simulink model "multifoc"  (R2025b)
settings: Solver=FixedStepAuto  StartTime=0.0  StopTime=inf  RelTol=1e-3
model workspace (MAT data in the model file):
  idx = Simulink.Parameter
  idx.Value = 15
  idx.Complexity = 'real'
  idx.Dimensions = [1 1]
  idx.DataType = 'auto'
undefined symbols (not defined in the file): AmcfocInitConf, ControlModes, EventTypes, externals, motor_id
libraries: simulink x4, dspsigops x2
settings Model: DataDictionary=amcfoc.sldd  SimulationMode=accelerator  Creator=mfussi  LastModifiedBy=rpumpo
settings SolverCC: ConcurrentTasks=on  AutoInsertRateTranBlk=on
settings DataIOCC: SaveOutput=off  DSMLogging=off  SaveTime=off
settings OptimizationCC: SimCompilerOptimization=on
settings RTWCC: GPUComputeCapability=3.5

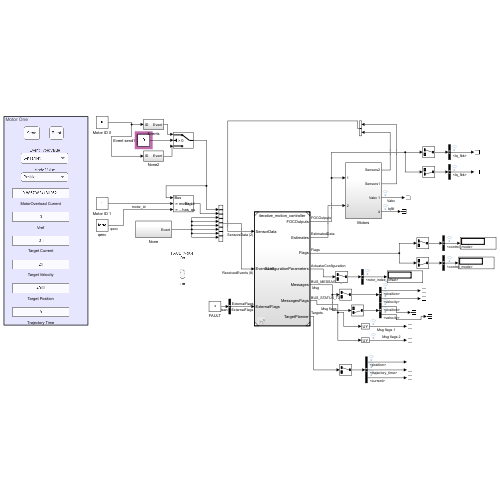
[thumbnail: Simulink's stored preview of the top-level diagram]
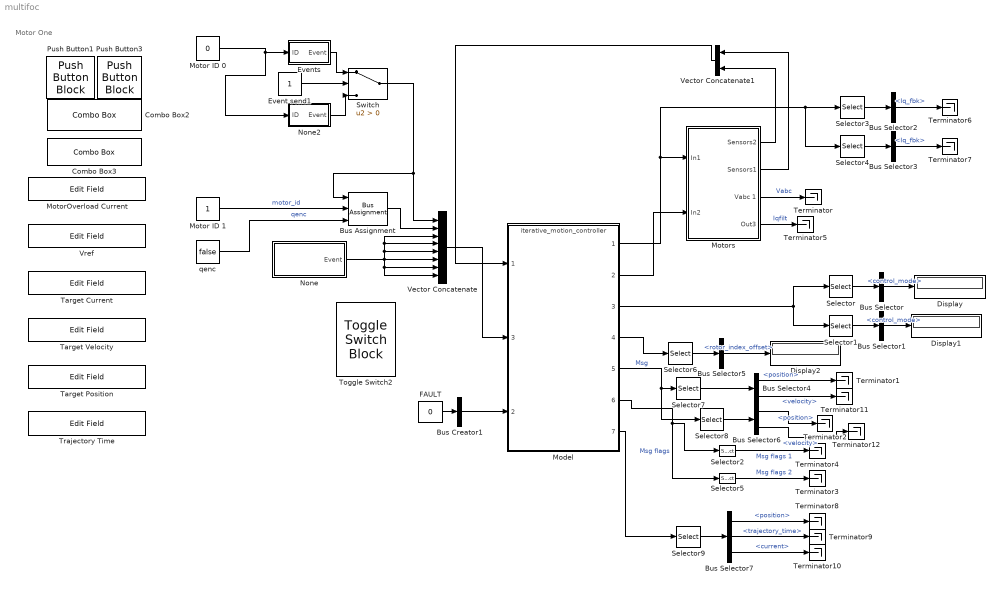
== system multifoc ==
  note: Motor One
  Bus Assignment : BusAssignment  AssignedSignals=motor_id,externals.has_quadrature_encoder
  Bus Creator1 : BusCreator  Inputs=1  OutDataTypeStr=Bus: ExternalFlags  NonVirtualBus=on
      settings: InheritFromInputs=off
  Bus Selector : BusSelector  OutputSignals=control_mode
  Bus Selector1 : BusSelector  OutputSignals=control_mode
  Bus Selector2 : BusSelector  OutputSignals=Iq_fbk
  Bus Selector3 : BusSelector  OutputSignals=Iq_fbk
  Bus Selector4 : BusSelector  OutputSignals=foc.position,foc.velocity
  Bus Selector5 : BusSelector  OutputSignals=motor.externals.rotor_index_offset
  Bus Selector6 : BusSelector  OutputSignals=foc.position,foc.velocity
  Bus Selector7 : BusSelector  OutputSignals=position,trajectory_time,current
  Combo Box2 : ComboBox  SelectedLabel=SetTarget  UseEnumeratedDataType=on  EnumeratedDataType=EventTypes
  Combo Box3 : ComboBox  SelectedLabel=Position  UseEnumeratedDataType=on  EnumeratedDataType=ControlModes
  Display : Display
  Display1 : Display
  Display2 : Display
  Event send1 : Constant
  Events : Subsystem
  FAULT : Constant  Value=0  OutDataTypeStr=Inherit: Inherit via back propagation
  Model : ModelReference  ModelNameDialog=iterative_motion_controller.slx  SimulationMode=Normal  ModelReferenceVersion=5.18
      settings: PortSchema="{\"entries\":[{\"content\":{\"sides\":[{\"content\":{\"connectorIds\":[\"In1\",\"In3\",\"In2\"]},\"type\":\"ConnectorPlacement.EquallySpacedRectSide\",\"uuid\":\"934c1d33-4450-4a0d-b709-1a42a1f76a8a\"},{\"content\":{\"connectorIds\":[\"Out1\",\"Out2\",\"Out3\",\"Out4\",\"Out5\",\"Out6\",\"Out7\"],\"side\":\"RIGHT\"},\"type\":\"ConnectorPlacement.EquallySpacedRectSide\",\"uuid\":\"07cc3f64-4a6c-4a49-ab3b-6bdd8946d703\"},{\"content\":{\"side\":\"TOP\"},\"type\":\"ConnectorPlacement.EquallySpacedRectSide\",\"uuid\":\"bdfb7dfb-875f-4552-909e-d1a15bca8e36\"}]},\"type\":\"ConnectorPlacement.EquallySpacedConnector\",\"uuid\":\"d809c882-6d9c-4cbc-bba4-fc08c365081a\"}],\"packageUris\":[\"http://schema.mathworks.com/mf0/Connector/R2020b\"],\"version\":\"1.0\"}"
  Motor ID 0 : Constant  Value=0  OutDataTypeStr=Inherit: Inherit via back propagation
  Motor ID 1 : Constant  OutDataTypeStr=Inherit: Inherit via back propagation
  MotorOverload Current : EditField  LabelPosition=Hide  ShowInitialText=on  Alignment=Center
  Motors : Subsystem
  None : Subsystem
  None2 : Subsystem
  Push Button1 : PushButtonBlock  ButtonText=Send  IconOnColor=[0.0, 0.39215686274509803, 0.0]  IconOffColor=[0.0, 1.0, 0.0]  OffValue=0.000000
  Push Button3 : PushButtonBlock  ButtonText=Burst  ButtonType=Latch  IconOnColor=[0.0, 0.39215686274509803, 0.0]  IconOffColor=[0.0, 1.0, 0.0]  OffValue=0.000000
  Selector{,2..3,6..7,9} (6 alike) : Selector  InputPortWidth=2  IndexOptions=Index vector (dialog)  Indices=1  OutputSizes=1
  Selector{1,4..5,8} (4 alike) : Selector  InputPortWidth=2  IndexOptions=Index vector (dialog)  Indices=2  OutputSizes=1
  Switch : Switch  Criteria=u2 > Threshold  SaturateOnIntegerOverflow=off  InputSameDT=off
  Target Current : EditField  LabelPosition=Hide  ShowInitialText=on  Alignment=Center
  Target Position : EditField  LabelPosition=Hide  ShowInitialText=on  Alignment=Center
  Target Velocity : EditField  LabelPosition=Hide  ShowInitialText=on  Alignment=Center
  Terminator{,1..12} (13 alike) : Terminator
  Toggle Switch2 : ToggleSwitchBlock
  Trajectory Time : EditField  LabelPosition=Hide  ShowInitialText=on  Alignment=Center
  Vector Concatenate : Concatenate  NumInputs=8
  Vector Concatenate1 : Concatenate
  Vref : EditField  LabelPosition=Hide  ShowInitialText=on  Alignment=Center
  qenc : Constant  Value=false  OutDataTypeStr=boolean
  wires:
  Event send1/1 -> Switch/2
  None/1(Event) -> Vector Concatenate/3, Vector Concatenate/4, Vector Concatenate/5, Vector Concatenate/8, Vector Concatenate/7, Vector Concatenate/6
  FAULT/1 -> Bus Creator1/1
  Bus Creator1/1 -> Model/2
  Vector Concatenate1/1 -> Model/1
  Motors/2(Sensors1) -> Vector Concatenate1/1
  Motors/3(Vabc 1) -> Terminator/1  "Vabc"
  Motors/4(Out3) -> Terminator5/1  "Iqfilt"
  Selector/1 -> Bus Selector/1
  Selector1/1 -> Bus Selector1/1
  Bus Selector/1 -> Display/1  "<control_mode>"
  Bus Selector1/1 -> Display1/1  "<control_mode>"
  Motors/1(Sensors2) -> Vector Concatenate1/2
  Model/1 -> Selector4/1, Selector3/1, Motors/1(In1)
  Bus Selector2/1 -> Terminator6/1  "<Iq_fbk>"
  Bus Selector3/1 -> Terminator7/1  "<Iq_fbk>"
  Selector4/1 -> Bus Selector3/1
  Selector3/1 -> Bus Selector2/1
  Model/2 -> Motors/2(In2)
  Model/6 -> Selector2/1, Selector5/1  "Msg flags"
  Model/5 -> Selector8/1, Selector7/1  "Msg"
  Selector5/1 -> Terminator3/1  "Msg flags 2"
  Selector2/1 -> Terminator4/1  "Msg flags 1"
  Motor ID 1/1 -> Bus Assignment/2  "motor_id"
  Motor ID 0/1 -> Events/1(ID), None2/1(ID)
  qenc/1 -> Bus Assignment/3  "qenc"
  Model/3 -> Selector/1, Selector1/1
  Model/4 -> Selector6/1
  Selector6/1 -> Bus Selector5/1
  Bus Selector5/1 -> Display2/1  "<rotor_index_offset>"
  Selector7/1 -> Bus Selector4/1
  Selector8/1 -> Bus Selector6/1
  Bus Selector4/1 -> Terminator1/1  "<position>"
  Bus Selector6/1 -> Terminator2/1  "<position>"
  Model/7 -> Selector9/1
  Selector9/1 -> Bus Selector7/1
  Bus Selector7/1 -> Terminator8/1  "<position>"
  Bus Selector7/2 -> Terminator9/1  "<trajectory_time>"
  Vector Concatenate/1 -> Model/3
  Events/1(Event) -> Switch/1
  Bus Selector7/3 -> Terminator10/1  "<current>"
  None2/1(Event) -> Switch/3
  Switch/1 -> Vector Concatenate/1, Bus Assignment/1
  Bus Assignment/1 -> Vector Concatenate/2
  Bus Selector4/2 -> Terminator11/1  "<velocity>"
  Bus Selector6/2 -> Terminator12/1  "<velocity>"

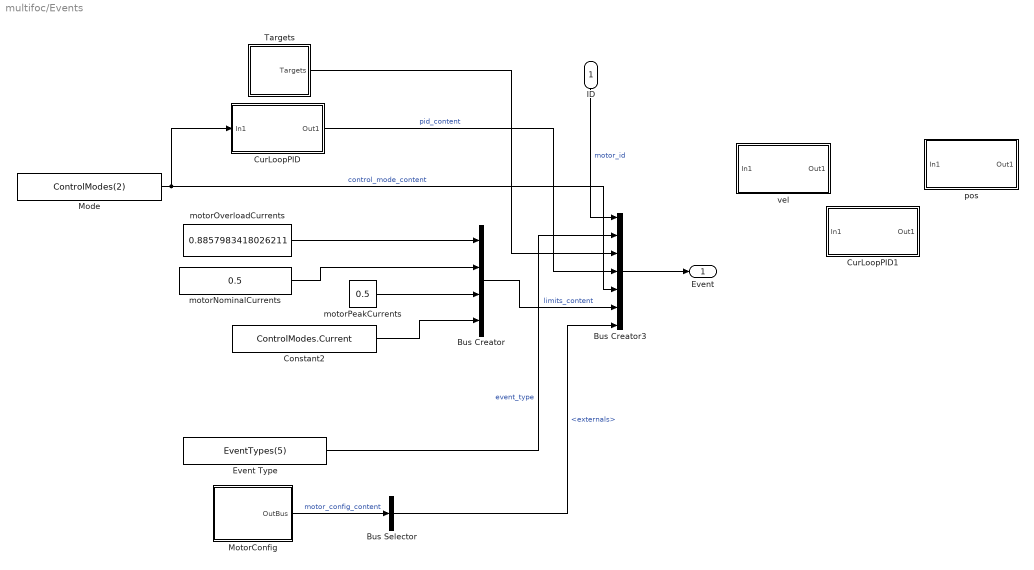
== system multifoc/Events ==
  ID : Inport
  Bus Creator : BusCreator  Inputs=4  OutDataTypeStr=Bus: SupervisorInputLimits
  Bus Creator3 : BusCreator  Inputs=7  OutDataTypeStr=Bus: ReceivedEvents  NonVirtualBus=on
  Bus Selector : BusSelector  OutputSignals=externals
  Constant2 : Constant  Value=ControlModes.Current  OutDataTypeStr=Enum: ControlModes
  CurLoopPID : Subsystem  mask{OutMax=3, OutMin=-3, P=10, I=10, D=0, N=0, I0=0, D0=0, shift_factor=0}
      mask prompts: shift_factor "Shift Factor"
  CurLoopPID1 : Subsystem  mask{OutMax=0, OutMin=0, P=2, I=500, D=0, N=10, I0=0, D0=0, shift_factor=0}
      mask prompts: shift_factor "Shift Factor"
  Event Type : Constant  Value=EventTypes(5)  OutDataTypeStr=Enum: EventTypes
  Mode : Constant  Value=ControlModes(2)  OutDataTypeStr=Enum: ControlModes
  MotorConfig : Subsystem  mask{has_hall_sens=AmcfocInitConf(1).motor.externals.has_hall_sens, has_quadrature_encoder=false, has_speed_quadrature_encoder=AmcfocInitConf(1).motor.externals.has_speed_quadrature_encoder, has_torque_sens=AmcfocInitConf(1).motor.externals.has_temperature_sens, use_index=false, enable_verbosity=AmcfocInitConf(1).motor.externals.enable_verbosity, hall_sensors_offset=0, rotor_encoder_resolution=1, rotor_index_offset=AmcfocInitConf(1).motor.externals.rotor_index_offset, encoder_tolerance=AmcfocInitConf(1).motor.externals.encoder_tolerance, pole_pairs=AmcfocInitConf(1).motor.externals.pole_pairs, reduction=100, Kbemf=AmcfocInitConf(1).motor.Kbemf, Rphase=AmcfocInitConf(1).motor.Rphase, Imin=AmcfocInitConf(1).motor.Imin, Imax=AmcfocInitConf(1).motor.Imax, Vmax=AmcfocInitConf(1).motor.Vmax, R=AmcfocInitConf(1).motor.resistance, L=AmcfocInitConf(1).motor.inductance, Rt=AmcfocInitConf(1).motor.thermal_resistance, tau=AmcfocInitConf(1).motor.thermal_time_constant}
      mask prompts: R "Motor Resistance"; L "Motor Inductance"; Rt "Thermal Resistance"; tau "Thermal Time Constant"
  Targets : Subsystem
  motorNominalCurrents : Constant  Value=0.5  OutDataTypeStr=single
  motorOverloadCurrents : Constant  Value=0.8857983418026211  OutDataTypeStr=single
  motorPeakCurrents : Constant  Value=0.5  OutDataTypeStr=single
  pos : Subsystem  mask{OutMax=0, OutMin=0, P=2, I=500, D=0, N=10, I0=0, D0=0, shift_factor=0}
      mask prompts: shift_factor "Shift Factor"
  vel : Subsystem  mask{OutMax=0, OutMin=0, P=2, I=500, D=0, N=10, I0=0, D0=0, shift_factor=0}
      mask prompts: shift_factor "Shift Factor"
  Event : Outport  OutDataTypeStr=Bus: ReceivedEvents
  wires:
  Bus Creator/1 -> Bus Creator3/6  "limits_content"
  Bus Selector/1 -> Bus Creator3/7  "<externals>"
  Mode/1 -> Bus Creator3/5, CurLoopPID/1(In1)  "control_mode_content"
  Event Type/1 -> Bus Creator3/2  "event_type"
  CurLoopPID/1(Out1) -> Bus Creator3/4  "pid_content"
  motorPeakCurrents/1 -> Bus Creator/3
  Constant2/1 -> Bus Creator/4
  motorOverloadCurrents/1 -> Bus Creator/1
  motorNominalCurrents/1 -> Bus Creator/2
  Bus Creator3/1 -> Event/1
  ID/1 -> Bus Creator3/1  "motor_id"
  MotorConfig/1(OutBus) -> Bus Selector/1  "motor_config_content"
  Targets/1(Targets) -> Bus Creator3/3

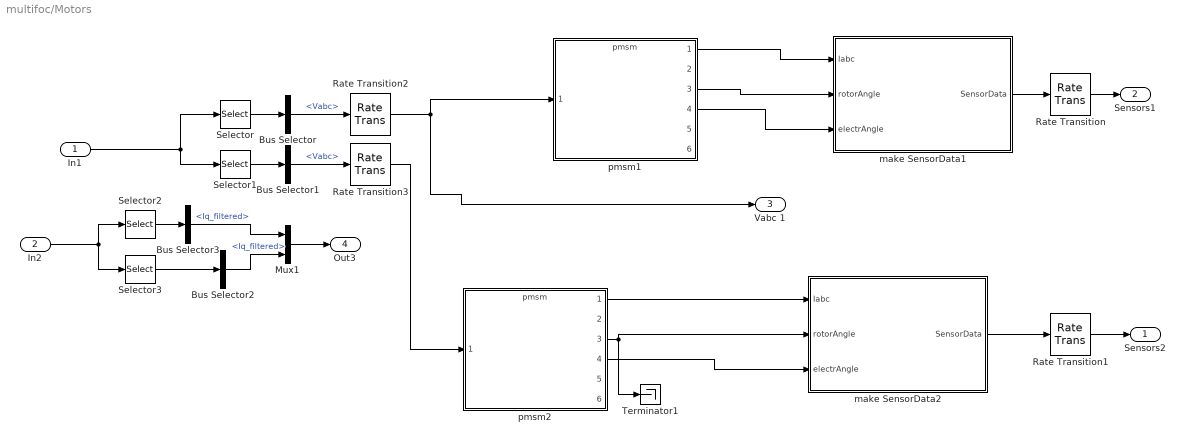
== system multifoc/Motors ==
  In1 : Inport
  In2 : Inport  Port=2
  Bus Selector : BusSelector  OutputSignals=Vabc
  Bus Selector1 : BusSelector  OutputSignals=Vabc
  Bus Selector2 : BusSelector  OutputSignals=Iq_filtered
  Bus Selector3 : BusSelector  OutputSignals=Iq_filtered
  Mux1 : Mux  Inputs=2
  Rate Transition : RateTransition  Integrity=off  OutPortSampleTime=Ts_ControlFOC
  Rate Transition1 : RateTransition  Integrity=off  OutPortSampleTime=Ts_ControlFOC
  Rate Transition2 : RateTransition  Integrity=off
  Rate Transition3 : RateTransition  Integrity=off
  Selector : Selector  InputPortWidth=2  IndexOptions=Index vector (dialog)  Indices=1  OutputSizes=1
  Selector1 : Selector  InputPortWidth=2  IndexOptions=Index vector (dialog)  Indices=2  OutputSizes=1
  Selector2 : Selector  InputPortWidth=2  IndexOptions=Index vector (dialog)  Indices=1  OutputSizes=1
  Selector3 : Selector  InputPortWidth=2  IndexOptions=Index vector (dialog)  Indices=2  OutputSizes=1
  Terminator1 : Terminator
  make SensorData1 : Subsystem
  make SensorData2 : Subsystem
  pmsm1 : ModelReference  ModelNameDialog=pmsm.slx  SimulationMode=Normal  ModelReferenceVersion=10.6  OutputSignalHandling=Zero-order hold
  pmsm2 : ModelReference  ModelNameDialog=pmsm.slx  SimulationMode=Normal  ModelReferenceVersion=10.6
  Sensors2 : Outport
  Sensors1 : Outport  Port=2
  Vabc 1 : Outport  Port=3
  Out3 : Outport  Port=4
  wires:
  pmsm2/1 -> make SensorData2/1(Iabc)
  Bus Selector1/1 -> Rate Transition3/1  "<Vabc>"
  make SensorData1/1(SensorData) -> Rate Transition/1
  Selector3/1 -> Bus Selector2/1
  pmsm2/3 -> make SensorData2/2(rotorAngle), Terminator1/1
  pmsm1/1 -> make SensorData1/1(Iabc)
  In2/1 -> Selector2/1, Selector3/1
  Bus Selector/1 -> Rate Transition2/1  "<Vabc>"
  Selector/1 -> Bus Selector/1
  Selector1/1 -> Bus Selector1/1
  Selector2/1 -> Bus Selector3/1
  Rate Transition2/1 -> pmsm1/1, Vabc 1/1
  Mux1/1 -> Out3/1
  make SensorData2/1(SensorData) -> Rate Transition1/1
  In1/1 -> Selector1/1, Selector/1
  Bus Selector3/1 -> Mux1/1  "<Iq_filtered>"
  Bus Selector2/1 -> Mux1/2  "<Iq_filtered>"
  Rate Transition/1 -> Sensors1/1
  Rate Transition1/1 -> Sensors2/1
  Rate Transition3/1 -> pmsm2/1
  pmsm1/3 -> make SensorData1/2(rotorAngle)
  pmsm1/4 -> make SensorData1/3(electrAngle)
  pmsm2/4 -> make SensorData2/3(electrAngle)

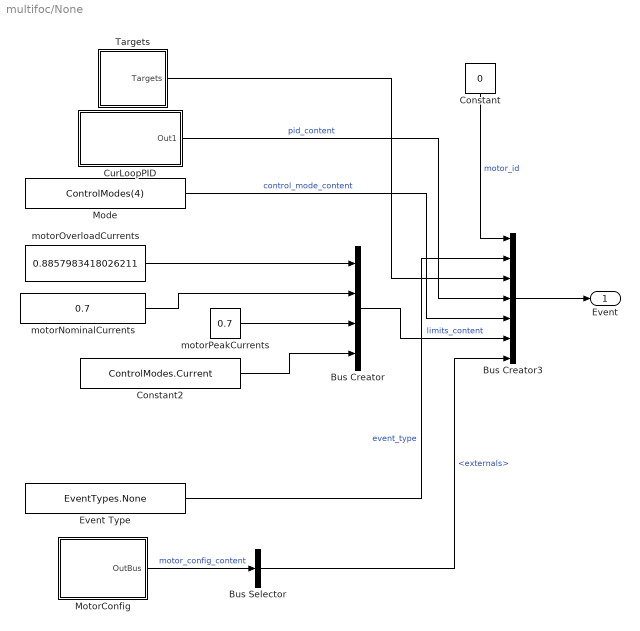
== system multifoc/None ==
  Bus Creator : BusCreator  Inputs=4  OutDataTypeStr=Bus: SupervisorInputLimits
  Bus Creator3 : BusCreator  Inputs=7  OutDataTypeStr=Bus: ReceivedEvents  NonVirtualBus=on
  Bus Selector : BusSelector  OutputSignals=externals
  Constant : Constant  Value=0  OutDataTypeStr=Inherit: Inherit via back propagation
  Constant2 : Constant  Value=ControlModes.Current  OutDataTypeStr=Enum: ControlModes
  CurLoopPID : Subsystem  mask{OutMax=0, OutMin=0, P=2, I=500, D=0, N=10, I0=0, D0=0, shift_factor=0}
      mask prompts: shift_factor "Shift Factor"
  Event Type : Constant  Value=EventTypes.None  OutDataTypeStr=Enum: EventTypes
  Mode : Constant  Value=ControlModes(4)  OutDataTypeStr=Enum: ControlModes
  MotorConfig : Subsystem  mask{has_hall_sens=AmcfocInitConf(1).motor.externals.has_hall_sens, has_quadrature_encoder=AmcfocInitConf(1).motor.externals.has_quadrature_encoder, has_speed_quadrature_encoder=AmcfocInitConf(1).motor.externals.has_speed_quadrature_encoder, has_torque_sens=AmcfocInitConf(1).motor.externals.has_temperature_sens, use_index=AmcfocInitConf(1).motor.externals.use_index, enable_verbosity=AmcfocInitConf(1).motor.externals.enable_verbosity, hall_sensors_offset=0, rotor_encoder_resolution=AmcfocInitConf(1).motor.externals.rotor_encoder_resolution, rotor_index_offset=AmcfocInitConf(1).motor.externals.rotor_index_offset, encoder_tolerance=AmcfocInitConf(1).motor.externals.encoder_tolerance, pole_pairs=AmcfocInitConf(1).motor.externals.pole_pairs, reduction=100, Kbemf=AmcfocInitConf(1).motor.Kbemf, Rphase=AmcfocInitConf(1).motor.Rphase, Imin=AmcfocInitConf(1).motor.Imin, Imax=AmcfocInitConf(1).motor.Imax, Vmax=AmcfocInitConf(1).motor.Vmax, R=AmcfocInitConf(1).motor.resistance, L=AmcfocInitConf(1).motor.inductance, Rt=AmcfocInitConf(1).motor.thermal_resistance, tau=AmcfocInitConf(1).motor.thermal_time_constant}
      mask prompts: R "Motor Resistance"; L "Motor Inductance"; Rt "Thermal Resistance"; tau "Thermal Time Constant"
  Targets : Subsystem
  motorNominalCurrents : Constant  Value=0.7  OutDataTypeStr=single
  motorOverloadCurrents : Constant  Value=0.8857983418026211  OutDataTypeStr=single
  motorPeakCurrents : Constant  Value=0.7  OutDataTypeStr=single
  Event : Outport  OutDataTypeStr=Bus: ReceivedEvents
  wires:
  Bus Creator/1 -> Bus Creator3/6  "limits_content"
  Bus Selector/1 -> Bus Creator3/7  "<externals>"
  Mode/1 -> Bus Creator3/5  "control_mode_content"
  Event Type/1 -> Bus Creator3/2  "event_type"
  CurLoopPID/1(Out1) -> Bus Creator3/4  "pid_content"
  motorPeakCurrents/1 -> Bus Creator/3
  Constant2/1 -> Bus Creator/4
  motorOverloadCurrents/1 -> Bus Creator/1
  motorNominalCurrents/1 -> Bus Creator/2
  Bus Creator3/1 -> Event/1
  Constant/1 -> Bus Creator3/1  "motor_id"
  MotorConfig/1(OutBus) -> Bus Selector/1  "motor_config_content"
  Targets/1(Targets) -> Bus Creator3/3

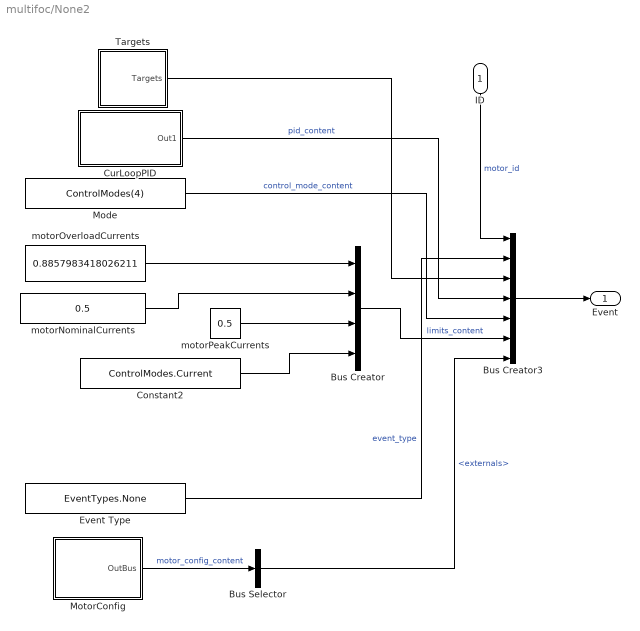
== system multifoc/None2 ==
  ID : Inport
  Bus Creator : BusCreator  Inputs=4  OutDataTypeStr=Bus: SupervisorInputLimits
  Bus Creator3 : BusCreator  Inputs=7  OutDataTypeStr=Bus: ReceivedEvents  NonVirtualBus=on
  Bus Selector : BusSelector  OutputSignals=externals
  Constant2 : Constant  Value=ControlModes.Current  OutDataTypeStr=Enum: ControlModes
  CurLoopPID : Subsystem  mask{OutMax=0, OutMin=0, P=0, I=0, D=0, N=10, I0=0, D0=0, shift_factor=0}
      mask prompts: shift_factor "Shift Factor"
  Event Type : Constant  Value=EventTypes.None  OutDataTypeStr=Enum: EventTypes
  Mode : Constant  Value=ControlModes(4)  OutDataTypeStr=Enum: ControlModes
  MotorConfig : Subsystem  mask{has_hall_sens=AmcfocInitConf(1).motor.externals.has_hall_sens, has_quadrature_encoder=true, has_speed_quadrature_encoder=AmcfocInitConf(1).motor.externals.has_speed_quadrature_encoder, has_torque_sens=AmcfocInitConf(1).motor.externals.has_temperature_sens, use_index=true, enable_verbosity=AmcfocInitConf(1).motor.externals.enable_verbosity, hall_sensors_offset=0, rotor_encoder_resolution=100, rotor_index_offset=AmcfocInitConf(1).motor.externals.rotor_index_offset, encoder_tolerance=AmcfocInitConf(1).motor.externals.encoder_tolerance, pole_pairs=AmcfocInitConf(1).motor.externals.pole_pairs, reduction=100, Kbemf=AmcfocInitConf(1).motor.Kbemf, Rphase=AmcfocInitConf(1).motor.Rphase, Imin=AmcfocInitConf(1).motor.Imin, Imax=AmcfocInitConf(1).motor.Imax, Vmax=AmcfocInitConf(1).motor.Vmax, R=AmcfocInitConf(1).motor.resistance, L=AmcfocInitConf(1).motor.inductance, Rt=AmcfocInitConf(1).motor.thermal_resistance, tau=AmcfocInitConf(1).motor.thermal_time_constant}
      mask prompts: R "Motor Resistance"; L "Motor Inductance"; Rt "Thermal Resistance"; tau "Thermal Time Constant"
  Targets : Subsystem
  motorNominalCurrents : Constant  Value=0.5  OutDataTypeStr=single
  motorOverloadCurrents : Constant  Value=0.8857983418026211  OutDataTypeStr=single
  motorPeakCurrents : Constant  Value=0.5  OutDataTypeStr=single
  Event : Outport  OutDataTypeStr=Bus: ReceivedEvents
  wires:
  Bus Creator/1 -> Bus Creator3/6  "limits_content"
  Bus Selector/1 -> Bus Creator3/7  "<externals>"
  Mode/1 -> Bus Creator3/5  "control_mode_content"
  Event Type/1 -> Bus Creator3/2  "event_type"
  CurLoopPID/1(Out1) -> Bus Creator3/4  "pid_content"
  motorPeakCurrents/1 -> Bus Creator/3
  Constant2/1 -> Bus Creator/4
  motorOverloadCurrents/1 -> Bus Creator/1
  motorNominalCurrents/1 -> Bus Creator/2
  Bus Creator3/1 -> Event/1
  ID/1 -> Bus Creator3/1  "motor_id"
  MotorConfig/1(OutBus) -> Bus Selector/1  "motor_config_content"
  Targets/1(Targets) -> Bus Creator3/3

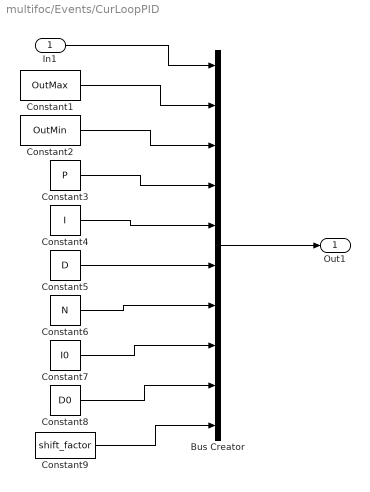
== system multifoc/Events/CurLoopPID ==
  In1 : Inport
  Bus Creator : BusCreator  Inputs=10  OutDataTypeStr=Bus: PID  NonVirtualBus=on
      settings: InheritFromInputs=off
  Constant1 : Constant  Value=OutMax  OutDataTypeStr=single
  Constant2 : Constant  Value=OutMin  OutDataTypeStr=single
  Constant3 : Constant  Value=P  OutDataTypeStr=single
  Constant4 : Constant  Value=I  OutDataTypeStr=single
  Constant5 : Constant  Value=D  OutDataTypeStr=single
  Constant6 : Constant  Value=N  OutDataTypeStr=single
  Constant7 : Constant  Value=I0  OutDataTypeStr=single
  Constant8 : Constant  Value=D0  OutDataTypeStr=single
  Constant9 : Constant  Value=shift_factor  OutDataTypeStr=uint8
  Out1 : Outport  OutDataTypeStr=Bus: PID
  wires:
  Bus Creator/1 -> Out1/1
  Constant8/1 -> Bus Creator/9
  Constant3/1 -> Bus Creator/4
  Constant5/1 -> Bus Creator/6
  Constant1/1 -> Bus Creator/2
  Constant7/1 -> Bus Creator/8
  Constant2/1 -> Bus Creator/3
  Constant9/1 -> Bus Creator/10
  Constant4/1 -> Bus Creator/5
  In1/1 -> Bus Creator/1
  Constant6/1 -> Bus Creator/7

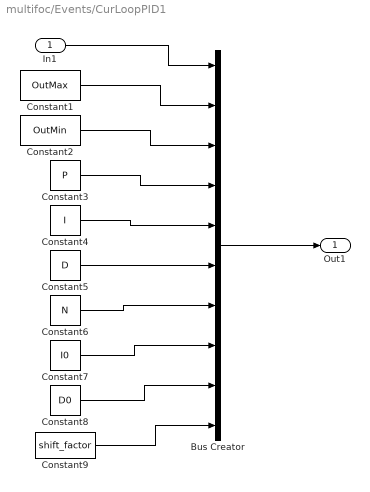
== system multifoc/Events/CurLoopPID1 ==
  In1 : Inport
  Bus Creator : BusCreator  Inputs=10  OutDataTypeStr=Bus: PID  NonVirtualBus=on
      settings: InheritFromInputs=off
  Constant1 : Constant  Value=OutMax  OutDataTypeStr=single
  Constant2 : Constant  Value=OutMin  OutDataTypeStr=single
  Constant3 : Constant  Value=P  OutDataTypeStr=single
  Constant4 : Constant  Value=I  OutDataTypeStr=single
  Constant5 : Constant  Value=D  OutDataTypeStr=single
  Constant6 : Constant  Value=N  OutDataTypeStr=single
  Constant7 : Constant  Value=I0  OutDataTypeStr=single
  Constant8 : Constant  Value=D0  OutDataTypeStr=single
  Constant9 : Constant  Value=shift_factor  OutDataTypeStr=uint8
  Out1 : Outport  OutDataTypeStr=Bus: PID
  wires:
  Bus Creator/1 -> Out1/1
  Constant8/1 -> Bus Creator/9
  Constant3/1 -> Bus Creator/4
  Constant5/1 -> Bus Creator/6
  Constant1/1 -> Bus Creator/2
  Constant7/1 -> Bus Creator/8
  Constant2/1 -> Bus Creator/3
  Constant9/1 -> Bus Creator/10
  Constant4/1 -> Bus Creator/5
  In1/1 -> Bus Creator/1
  Constant6/1 -> Bus Creator/7

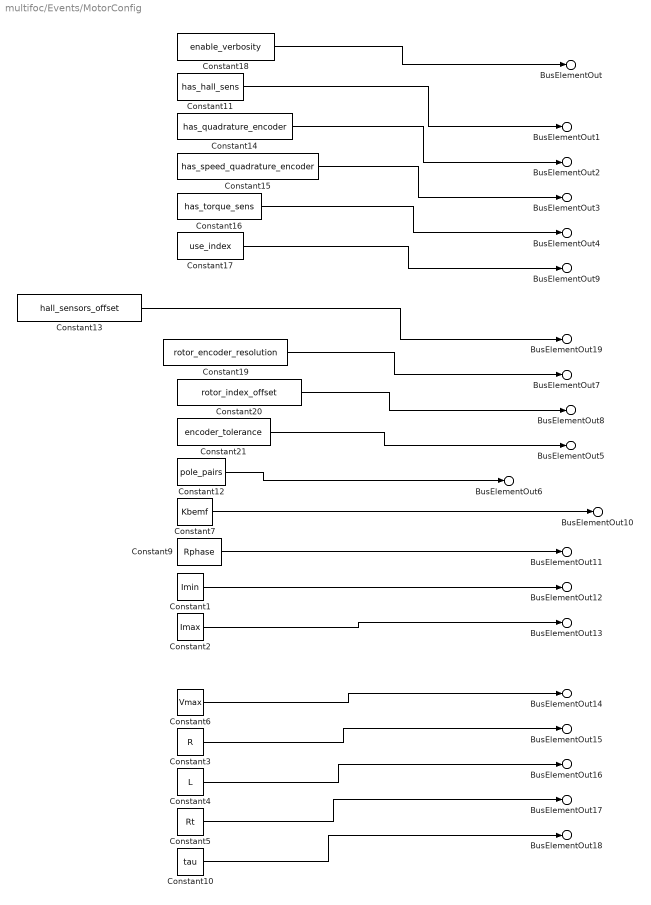
== system multifoc/Events/MotorConfig ==
  Constant1 : Constant  Value=Imin  OutDataTypeStr=single
  Constant10 : Constant  Value=tau  OutDataTypeStr=single
  Constant11 : Constant  Value=has_hall_sens  OutDataTypeStr=boolean
  Constant12 : Constant  Value=pole_pairs  OutDataTypeStr=uint8
  Constant13 : Constant  Value=hall_sensors_offset  OutDataTypeStr=Inherit: Inherit via back propagation
  Constant14 : Constant  Value=has_quadrature_encoder  OutDataTypeStr=boolean
  Constant15 : Constant  Value=has_speed_quadrature_encoder  OutDataTypeStr=boolean
  Constant16 : Constant  Value=has_torque_sens  OutDataTypeStr=boolean
  Constant17 : Constant  Value=use_index  OutDataTypeStr=boolean
  Constant18 : Constant  Value=enable_verbosity  OutDataTypeStr=boolean
  Constant19 : Constant  Value=rotor_encoder_resolution  OutDataTypeStr=int16
  Constant2 : Constant  Value=Imax  OutDataTypeStr=single
  Constant20 : Constant  Value=rotor_index_offset  OutDataTypeStr=int16
  Constant21 : Constant  Value=encoder_tolerance  OutDataTypeStr=uint8
  Constant3 : Constant  Value=R  OutDataTypeStr=single
  Constant4 : Constant  Value=L  OutDataTypeStr=single
  Constant5 : Constant  Value=Rt  OutDataTypeStr=single
  Constant6 : Constant  Value=Vmax  OutDataTypeStr=single
  Constant7 : Constant  Value=Kbemf  OutDataTypeStr=single
  Constant9 : Constant  Value=Rphase  OutDataTypeStr=single
  BusElementOut : Outport  PortName=OutBus  Element=externals.enable_verbosity
  BusElementOut1 : Outport  PortName=OutBus  Element=externals.has_hall_sens
  BusElementOut2 : Outport  PortName=OutBus  Element=externals.has_quadrature_encoder
  BusElementOut3 : Outport  PortName=OutBus  Element=externals.has_speed_quadrature_encoder
  BusElementOut4 : Outport  PortName=OutBus  Element=externals.has_temperature_sens
  BusElementOut5 : Outport  PortName=OutBus  Element=externals.encoder_tolerance
  BusElementOut6 : Outport  PortName=OutBus  Element=externals.pole_pairs
  BusElementOut7 : Outport  PortName=OutBus  Element=externals.rotor_encoder_resolution
  BusElementOut8 : Outport  PortName=OutBus  Element=externals.rotor_index_offset
  BusElementOut9 : Outport  PortName=OutBus  Element=externals.use_index
  BusElementOut10 : Outport  PortName=OutBus  Element=Kbemf
  BusElementOut11 : Outport  PortName=OutBus  Element=Rphase
  BusElementOut12 : Outport  PortName=OutBus  Element=Imin
  BusElementOut13 : Outport  PortName=OutBus  Element=Imax
  BusElementOut14 : Outport  PortName=OutBus  Element=Vmax
  BusElementOut15 : Outport  PortName=OutBus  Element=resistance
  BusElementOut16 : Outport  PortName=OutBus  Element=inductance
  BusElementOut17 : Outport  PortName=OutBus  Element=thermal_resistance
  BusElementOut18 : Outport  PortName=OutBus  Element=thermal_time_constant
  BusElementOut19 : Outport  PortName=OutBus  Element=hall_sensors_offset
  wires:
  Constant15/1 -> BusElementOut3/1
  Constant18/1 -> BusElementOut/1
  Constant14/1 -> BusElementOut2/1
  Constant16/1 -> BusElementOut4/1
  Constant17/1 -> BusElementOut9/1
  Constant11/1 -> BusElementOut1/1
  Constant13/1 -> BusElementOut19/1
  Constant1/1 -> BusElementOut12/1
  Constant10/1 -> BusElementOut18/1
  Constant5/1 -> BusElementOut17/1
  Constant20/1 -> BusElementOut8/1
  Constant4/1 -> BusElementOut16/1
  Constant3/1 -> BusElementOut15/1
  Constant7/1 -> BusElementOut10/1
  Constant12/1 -> BusElementOut6/1
  Constant9/1 -> BusElementOut11/1
  Constant2/1 -> BusElementOut13/1
  Constant19/1 -> BusElementOut7/1
  Constant21/1 -> BusElementOut5/1
  Constant6/1 -> BusElementOut14/1

== system multifoc/Events/Targets ==
  Bus Creator : BusCreator  Inputs=5  OutDataTypeStr=Bus: Targets  NonVirtualBus=on
      settings: InheritFromInputs=off
  Data Type Conversion : DataTypeConversion  OutDataTypeStr=single  SaturateOnIntegerOverflow=off  RndMeth=Floor
  Data Type Conversion1 : DataTypeConversion  OutDataTypeStr=single  SaturateOnIntegerOverflow=off  RndMeth=Floor
  Trajectory Time : Constant  Value=2  OutDataTypeStr=single
  current Target : Constant  Value=-0.1
  jointposition : Constant  Value=4000  OutDataTypeStr=single
  jointvelocity : Constant  Value=20  OutDataTypeStr=single
  vref : Constant  Value=0  OutDataTypeStr=single
  Targets : Outport
  wires:
  Data Type Conversion1/1 -> Bus Creator/5
  Trajectory Time/1 -> Bus Creator/1
  jointposition/1 -> Bus Creator/2
  current Target/1 -> Data Type Conversion/1
  jointvelocity/1 -> Bus Creator/3
  vref/1 -> Data Type Conversion1/1
  Data Type Conversion/1 -> Bus Creator/4  "motorcurrent"
  Bus Creator/1 -> Targets/1

== system multifoc/Events/pos ==
  In1 : Inport
  Bus Creator : BusCreator  Inputs=10  OutDataTypeStr=Bus: PID  NonVirtualBus=on
      settings: InheritFromInputs=off
  Constant1 : Constant  Value=OutMax  OutDataTypeStr=single
  Constant2 : Constant  Value=OutMin  OutDataTypeStr=single
  Constant3 : Constant  Value=P  OutDataTypeStr=single
  Constant4 : Constant  Value=I  OutDataTypeStr=single
  Constant5 : Constant  Value=D  OutDataTypeStr=single
  Constant6 : Constant  Value=N  OutDataTypeStr=single
  Constant7 : Constant  Value=I0  OutDataTypeStr=single
  Constant8 : Constant  Value=D0  OutDataTypeStr=single
  Constant9 : Constant  Value=shift_factor  OutDataTypeStr=uint8
  Out1 : Outport  OutDataTypeStr=Bus: PID
  wires:
  Bus Creator/1 -> Out1/1
  Constant8/1 -> Bus Creator/9
  Constant3/1 -> Bus Creator/4
  Constant5/1 -> Bus Creator/6
  Constant1/1 -> Bus Creator/2
  Constant7/1 -> Bus Creator/8
  Constant2/1 -> Bus Creator/3
  Constant9/1 -> Bus Creator/10
  Constant4/1 -> Bus Creator/5
  In1/1 -> Bus Creator/1
  Constant6/1 -> Bus Creator/7

== system multifoc/Events/vel ==
  In1 : Inport
  Bus Creator : BusCreator  Inputs=10  OutDataTypeStr=Bus: PID  NonVirtualBus=on
      settings: InheritFromInputs=off
  Constant1 : Constant  Value=OutMax  OutDataTypeStr=single
  Constant2 : Constant  Value=OutMin  OutDataTypeStr=single
  Constant3 : Constant  Value=P  OutDataTypeStr=single
  Constant4 : Constant  Value=I  OutDataTypeStr=single
  Constant5 : Constant  Value=D  OutDataTypeStr=single
  Constant6 : Constant  Value=N  OutDataTypeStr=single
  Constant7 : Constant  Value=I0  OutDataTypeStr=single
  Constant8 : Constant  Value=D0  OutDataTypeStr=single
  Constant9 : Constant  Value=shift_factor  OutDataTypeStr=uint8
  Out1 : Outport  OutDataTypeStr=Bus: PID
  wires:
  Bus Creator/1 -> Out1/1
  Constant8/1 -> Bus Creator/9
  Constant3/1 -> Bus Creator/4
  Constant5/1 -> Bus Creator/6
  Constant1/1 -> Bus Creator/2
  Constant7/1 -> Bus Creator/8
  Constant2/1 -> Bus Creator/3
  Constant9/1 -> Bus Creator/10
  Constant4/1 -> Bus Creator/5
  In1/1 -> Bus Creator/1
  Constant6/1 -> Bus Creator/7

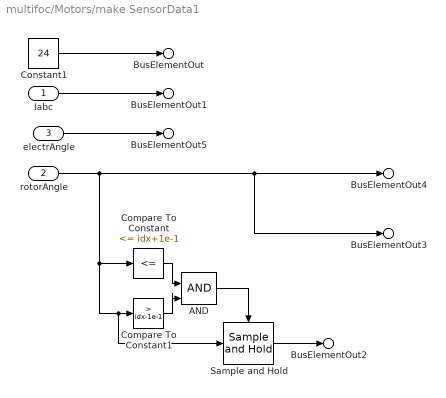
== system multifoc/Motors/make SensorData1 ==
  Iabc : Inport
  rotorAngle : Inport  Port=2
  electrAngle : Inport  Port=3
  AND : Logic  IconShape=distinctive  AllPortsSameDT=off  OutDataTypeStr=boolean
  Compare To Constant : simulink/Logic and Bit Operations/Compare To Constant  relop=<=  const=idx+1e-1  OutDataTypeStr=boolean
  Compare To Constant1 : simulink/Logic and Bit Operations/Compare To Constant  relop=>  const=idx-1e-1  OutDataTypeStr=boolean
  Constant1 : Constant  Value=24  OutDataTypeStr=Inherit: Inherit via back propagation
  Sample and Hold : dspsigops/Sample and Hold  trig=Rising edge  initCond=0  latchinput=off
  BusElementOut : Outport  Description=power supply voltage  PortName=SensorData  Element=driversensors.Vcc
  BusElementOut3 : Outport  Description=Mechanical Angle before gearbox  PortName=SensorData  Element=motorsensors.qencoder.rotor_angle
  BusElementOut4 : Outport  Description=Counter of the QENC  PortName=SensorData  Element=motorsensors.qencoder.counter
  BusElementOut2 : Outport  Description=Last QENC count where the index has been detected  PortName=SensorData  Element=motorsensors.qencoder.Idx_counter
  BusElementOut1 : Outport  PortName=SensorData  Element=motorsensors.Iabc
  BusElementOut5 : Outport  Description=electrical angle = angle * pole_pairs  PortName=SensorData  Element=motorsensors.electrical_angle
  wires:
  Constant1/1 -> BusElementOut/1
  Iabc/1 -> BusElementOut1/1
  Compare To Constant/1 -> AND/1
  Compare To Constant1/1 -> AND/2
  AND/1 -> Sample and Hold/Trigger
  Sample and Hold/1 -> BusElementOut2/1
  electrAngle/1 -> BusElementOut5/1
  rotorAngle/1 -> BusElementOut3/1, BusElementOut4/1, Sample and Hold/1, Compare To Constant1/1, Compare To Constant/1

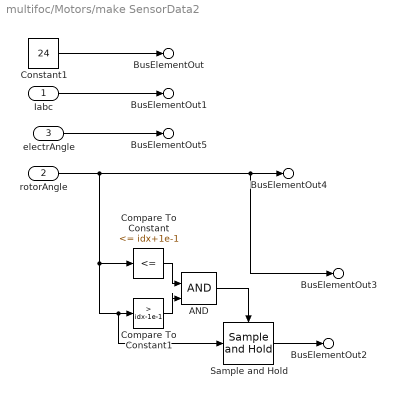
== system multifoc/Motors/make SensorData2 ==
  Iabc : Inport
  rotorAngle : Inport  Port=2
  electrAngle : Inport  Port=3
  AND : Logic  IconShape=distinctive  AllPortsSameDT=off  OutDataTypeStr=boolean
  Compare To Constant : simulink/Logic and Bit Operations/Compare To Constant  relop=<=  const=idx+1e-1  OutDataTypeStr=boolean
  Compare To Constant1 : simulink/Logic and Bit Operations/Compare To Constant  relop=>  const=idx-1e-1  OutDataTypeStr=boolean
  Constant1 : Constant  Value=24  OutDataTypeStr=Inherit: Inherit via back propagation
  Sample and Hold : dspsigops/Sample and Hold  trig=Rising edge  initCond=0  latchinput=off
  BusElementOut : Outport  Description=power supply voltage  PortName=SensorData  Element=driversensors.Vcc
  BusElementOut3 : Outport  Description=Mechanical Angle before gearbox  PortName=SensorData  Element=motorsensors.qencoder.rotor_angle
  BusElementOut4 : Outport  Description=Counter of the QENC  PortName=SensorData  Element=motorsensors.qencoder.counter
  BusElementOut2 : Outport  Description=Last QENC count where the index has been detected  PortName=SensorData  Element=motorsensors.qencoder.Idx_counter
  BusElementOut1 : Outport  PortName=SensorData  Element=motorsensors.Iabc
  BusElementOut5 : Outport  Description=electrical angle = angle * pole_pairs  PortName=SensorData  Element=motorsensors.electrical_angle
  wires:
  electrAngle/1 -> BusElementOut5/1
  AND/1 -> Sample and Hold/Trigger
  Compare To Constant1/1 -> AND/2
  Sample and Hold/1 -> BusElementOut2/1
  Iabc/1 -> BusElementOut1/1
  Constant1/1 -> BusElementOut/1
  Compare To Constant/1 -> AND/1
  rotorAngle/1 -> Sample and Hold/1, Compare To Constant1/1, Compare To Constant/1, BusElementOut3/1, BusElementOut4/1

== system multifoc/None/CurLoopPID ==
  Bus Creator : BusCreator  Inputs=10  OutDataTypeStr=Bus: PID  NonVirtualBus=on
      settings: InheritFromInputs=off
  Constant : Constant  Value=ControlModes.Current
  Constant1 : Constant  Value=OutMax  OutDataTypeStr=single
  Constant2 : Constant  Value=OutMin  OutDataTypeStr=single
  Constant3 : Constant  Value=P  OutDataTypeStr=single
  Constant4 : Constant  Value=I  OutDataTypeStr=single
  Constant5 : Constant  Value=D  OutDataTypeStr=single
  Constant6 : Constant  Value=N  OutDataTypeStr=single
  Constant7 : Constant  Value=I0  OutDataTypeStr=single
  Constant8 : Constant  Value=D0  OutDataTypeStr=single
  Constant9 : Constant  Value=shift_factor  OutDataTypeStr=uint8
  Out1 : Outport  OutDataTypeStr=Bus: PID
  wires:
  Bus Creator/1 -> Out1/1
  Constant8/1 -> Bus Creator/9
  Constant3/1 -> Bus Creator/4
  Constant5/1 -> Bus Creator/6
  Constant1/1 -> Bus Creator/2
  Constant7/1 -> Bus Creator/8
  Constant2/1 -> Bus Creator/3
  Constant9/1 -> Bus Creator/10
  Constant4/1 -> Bus Creator/5
  Constant/1 -> Bus Creator/1
  Constant6/1 -> Bus Creator/7

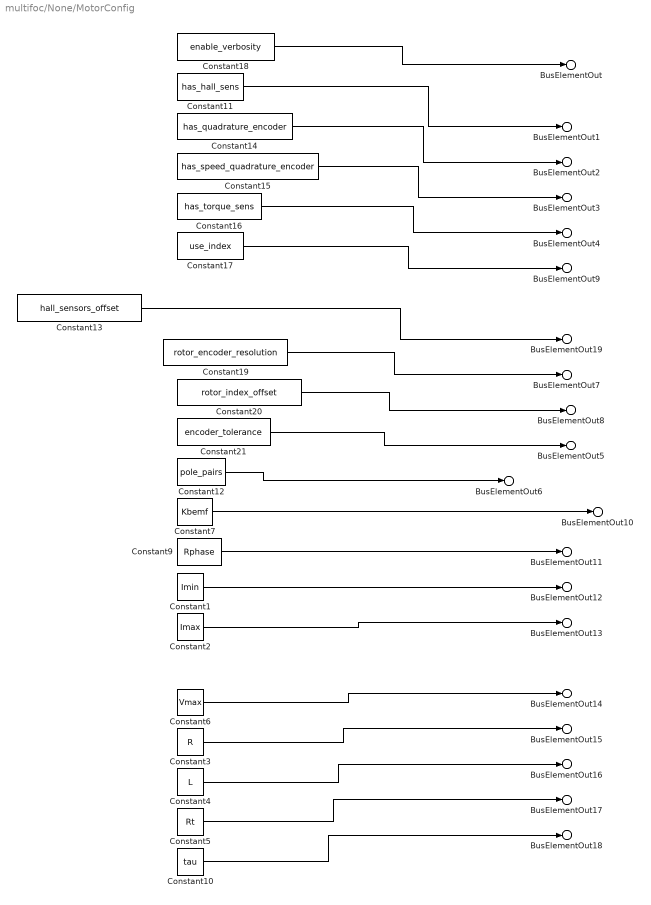
== system multifoc/None/MotorConfig ==
  Constant1 : Constant  Value=Imin  OutDataTypeStr=single
  Constant10 : Constant  Value=tau  OutDataTypeStr=single
  Constant11 : Constant  Value=has_hall_sens  OutDataTypeStr=boolean
  Constant12 : Constant  Value=pole_pairs  OutDataTypeStr=uint8
  Constant13 : Constant  Value=hall_sensors_offset  OutDataTypeStr=Inherit: Inherit via back propagation
  Constant14 : Constant  Value=has_quadrature_encoder  OutDataTypeStr=boolean
  Constant15 : Constant  Value=has_speed_quadrature_encoder  OutDataTypeStr=boolean
  Constant16 : Constant  Value=has_torque_sens  OutDataTypeStr=boolean
  Constant17 : Constant  Value=use_index  OutDataTypeStr=boolean
  Constant18 : Constant  Value=enable_verbosity  OutDataTypeStr=boolean
  Constant19 : Constant  Value=rotor_encoder_resolution  OutDataTypeStr=int16
  Constant2 : Constant  Value=Imax  OutDataTypeStr=single
  Constant20 : Constant  Value=rotor_index_offset  OutDataTypeStr=int16
  Constant21 : Constant  Value=encoder_tolerance  OutDataTypeStr=uint8
  Constant3 : Constant  Value=R  OutDataTypeStr=single
  Constant4 : Constant  Value=L  OutDataTypeStr=single
  Constant5 : Constant  Value=Rt  OutDataTypeStr=single
  Constant6 : Constant  Value=Vmax  OutDataTypeStr=single
  Constant7 : Constant  Value=Kbemf  OutDataTypeStr=single
  Constant9 : Constant  Value=Rphase  OutDataTypeStr=single
  BusElementOut : Outport  PortName=OutBus  Element=externals.enable_verbosity
  BusElementOut1 : Outport  PortName=OutBus  Element=externals.has_hall_sens
  BusElementOut2 : Outport  PortName=OutBus  Element=externals.has_quadrature_encoder
  BusElementOut3 : Outport  PortName=OutBus  Element=externals.has_speed_quadrature_encoder
  BusElementOut4 : Outport  PortName=OutBus  Element=externals.has_temperature_sens
  BusElementOut5 : Outport  PortName=OutBus  Element=externals.encoder_tolerance
  BusElementOut6 : Outport  PortName=OutBus  Element=externals.pole_pairs
  BusElementOut7 : Outport  PortName=OutBus  Element=externals.rotor_encoder_resolution
  BusElementOut8 : Outport  PortName=OutBus  Element=externals.rotor_index_offset
  BusElementOut9 : Outport  PortName=OutBus  Element=externals.use_index
  BusElementOut10 : Outport  PortName=OutBus  Element=Kbemf
  BusElementOut11 : Outport  PortName=OutBus  Element=Rphase
  BusElementOut12 : Outport  PortName=OutBus  Element=Imin
  BusElementOut13 : Outport  PortName=OutBus  Element=Imax
  BusElementOut14 : Outport  PortName=OutBus  Element=Vmax
  BusElementOut15 : Outport  PortName=OutBus  Element=resistance
  BusElementOut16 : Outport  PortName=OutBus  Element=inductance
  BusElementOut17 : Outport  PortName=OutBus  Element=thermal_resistance
  BusElementOut18 : Outport  PortName=OutBus  Element=thermal_time_constant
  BusElementOut19 : Outport  PortName=OutBus  Element=hall_sensors_offset
  wires:
  Constant15/1 -> BusElementOut3/1
  Constant18/1 -> BusElementOut/1
  Constant14/1 -> BusElementOut2/1
  Constant16/1 -> BusElementOut4/1
  Constant17/1 -> BusElementOut9/1
  Constant11/1 -> BusElementOut1/1
  Constant13/1 -> BusElementOut19/1
  Constant1/1 -> BusElementOut12/1
  Constant10/1 -> BusElementOut18/1
  Constant5/1 -> BusElementOut17/1
  Constant20/1 -> BusElementOut8/1
  Constant4/1 -> BusElementOut16/1
  Constant3/1 -> BusElementOut15/1
  Constant7/1 -> BusElementOut10/1
  Constant12/1 -> BusElementOut6/1
  Constant9/1 -> BusElementOut11/1
  Constant2/1 -> BusElementOut13/1
  Constant19/1 -> BusElementOut7/1
  Constant21/1 -> BusElementOut5/1
  Constant6/1 -> BusElementOut14/1

== system multifoc/None/Targets ==
  Bus Creator : BusCreator  Inputs=5  OutDataTypeStr=Bus: Targets  NonVirtualBus=on
      settings: InheritFromInputs=off
  Data Type Conversion : DataTypeConversion  OutDataTypeStr=single  SaturateOnIntegerOverflow=off  RndMeth=Floor
  Data Type Conversion1 : DataTypeConversion  OutDataTypeStr=single  SaturateOnIntegerOverflow=off  RndMeth=Floor
  Trajectory Time : Constant  Value=0  OutDataTypeStr=single
  current Target : Constant  Value=0.3342925916020326
  jointposition : Constant  Value=0  OutDataTypeStr=single
  jointvelocity : Constant  Value=0  OutDataTypeStr=single
  vref : Constant  Value=0  OutDataTypeStr=single
  Targets : Outport
  wires:
  Data Type Conversion1/1 -> Bus Creator/5
  Trajectory Time/1 -> Bus Creator/1
  jointposition/1 -> Bus Creator/2
  current Target/1 -> Data Type Conversion/1
  jointvelocity/1 -> Bus Creator/3
  vref/1 -> Data Type Conversion1/1
  Data Type Conversion/1 -> Bus Creator/4  "motorcurrent"
  Bus Creator/1 -> Targets/1

== system multifoc/None2/CurLoopPID ==
  Bus Creator : BusCreator  Inputs=10  OutDataTypeStr=Bus: PID  NonVirtualBus=on
      settings: InheritFromInputs=off
  Constant : Constant  Value=ControlModes.Current
  Constant1 : Constant  Value=OutMax  OutDataTypeStr=single
  Constant2 : Constant  Value=OutMin  OutDataTypeStr=single
  Constant3 : Constant  Value=P  OutDataTypeStr=single
  Constant4 : Constant  Value=I  OutDataTypeStr=single
  Constant5 : Constant  Value=D  OutDataTypeStr=single
  Constant6 : Constant  Value=N  OutDataTypeStr=single
  Constant7 : Constant  Value=I0  OutDataTypeStr=single
  Constant8 : Constant  Value=D0  OutDataTypeStr=single
  Constant9 : Constant  Value=shift_factor  OutDataTypeStr=uint8
  Out1 : Outport  OutDataTypeStr=Bus: PID
  wires:
  Bus Creator/1 -> Out1/1
  Constant8/1 -> Bus Creator/9
  Constant3/1 -> Bus Creator/4
  Constant5/1 -> Bus Creator/6
  Constant1/1 -> Bus Creator/2
  Constant7/1 -> Bus Creator/8
  Constant2/1 -> Bus Creator/3
  Constant9/1 -> Bus Creator/10
  Constant4/1 -> Bus Creator/5
  Constant/1 -> Bus Creator/1
  Constant6/1 -> Bus Creator/7

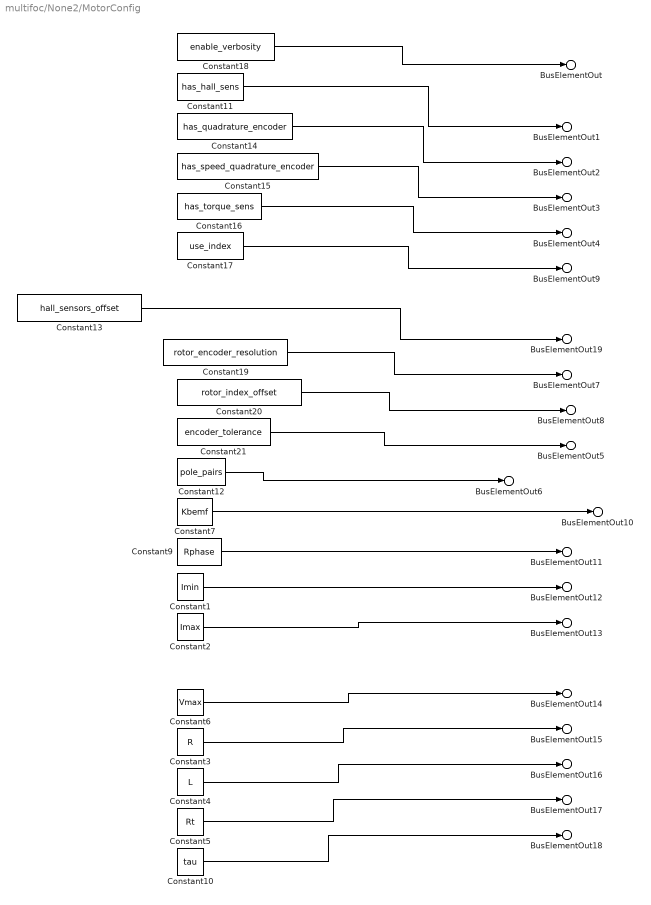
== system multifoc/None2/MotorConfig ==
  Constant1 : Constant  Value=Imin  OutDataTypeStr=single
  Constant10 : Constant  Value=tau  OutDataTypeStr=single
  Constant11 : Constant  Value=has_hall_sens  OutDataTypeStr=boolean
  Constant12 : Constant  Value=pole_pairs  OutDataTypeStr=uint8
  Constant13 : Constant  Value=hall_sensors_offset  OutDataTypeStr=Inherit: Inherit via back propagation
  Constant14 : Constant  Value=has_quadrature_encoder  OutDataTypeStr=boolean
  Constant15 : Constant  Value=has_speed_quadrature_encoder  OutDataTypeStr=boolean
  Constant16 : Constant  Value=has_torque_sens  OutDataTypeStr=boolean
  Constant17 : Constant  Value=use_index  OutDataTypeStr=boolean
  Constant18 : Constant  Value=enable_verbosity  OutDataTypeStr=boolean
  Constant19 : Constant  Value=rotor_encoder_resolution  OutDataTypeStr=int16
  Constant2 : Constant  Value=Imax  OutDataTypeStr=single
  Constant20 : Constant  Value=rotor_index_offset  OutDataTypeStr=int16
  Constant21 : Constant  Value=encoder_tolerance  OutDataTypeStr=uint8
  Constant3 : Constant  Value=R  OutDataTypeStr=single
  Constant4 : Constant  Value=L  OutDataTypeStr=single
  Constant5 : Constant  Value=Rt  OutDataTypeStr=single
  Constant6 : Constant  Value=Vmax  OutDataTypeStr=single
  Constant7 : Constant  Value=Kbemf  OutDataTypeStr=single
  Constant9 : Constant  Value=Rphase  OutDataTypeStr=single
  BusElementOut : Outport  PortName=OutBus  Element=externals.enable_verbosity
  BusElementOut1 : Outport  PortName=OutBus  Element=externals.has_hall_sens
  BusElementOut2 : Outport  PortName=OutBus  Element=externals.has_quadrature_encoder
  BusElementOut3 : Outport  PortName=OutBus  Element=externals.has_speed_quadrature_encoder
  BusElementOut4 : Outport  PortName=OutBus  Element=externals.has_temperature_sens
  BusElementOut5 : Outport  PortName=OutBus  Element=externals.encoder_tolerance
  BusElementOut6 : Outport  PortName=OutBus  Element=externals.pole_pairs
  BusElementOut7 : Outport  PortName=OutBus  Element=externals.rotor_encoder_resolution
  BusElementOut8 : Outport  PortName=OutBus  Element=externals.rotor_index_offset
  BusElementOut9 : Outport  PortName=OutBus  Element=externals.use_index
  BusElementOut10 : Outport  PortName=OutBus  Element=Kbemf
  BusElementOut11 : Outport  PortName=OutBus  Element=Rphase
  BusElementOut12 : Outport  PortName=OutBus  Element=Imin
  BusElementOut13 : Outport  PortName=OutBus  Element=Imax
  BusElementOut14 : Outport  PortName=OutBus  Element=Vmax
  BusElementOut15 : Outport  PortName=OutBus  Element=resistance
  BusElementOut16 : Outport  PortName=OutBus  Element=inductance
  BusElementOut17 : Outport  PortName=OutBus  Element=thermal_resistance
  BusElementOut18 : Outport  PortName=OutBus  Element=thermal_time_constant
  BusElementOut19 : Outport  PortName=OutBus  Element=hall_sensors_offset
  wires:
  Constant15/1 -> BusElementOut3/1
  Constant18/1 -> BusElementOut/1
  Constant14/1 -> BusElementOut2/1
  Constant16/1 -> BusElementOut4/1
  Constant17/1 -> BusElementOut9/1
  Constant11/1 -> BusElementOut1/1
  Constant13/1 -> BusElementOut19/1
  Constant1/1 -> BusElementOut12/1
  Constant10/1 -> BusElementOut18/1
  Constant5/1 -> BusElementOut17/1
  Constant20/1 -> BusElementOut8/1
  Constant4/1 -> BusElementOut16/1
  Constant3/1 -> BusElementOut15/1
  Constant7/1 -> BusElementOut10/1
  Constant12/1 -> BusElementOut6/1
  Constant9/1 -> BusElementOut11/1
  Constant2/1 -> BusElementOut13/1
  Constant19/1 -> BusElementOut7/1
  Constant21/1 -> BusElementOut5/1
  Constant6/1 -> BusElementOut14/1

== system multifoc/None2/Targets ==
  Bus Creator : BusCreator  Inputs=5  OutDataTypeStr=Bus: Targets  NonVirtualBus=on
      settings: InheritFromInputs=off
  Data Type Conversion : DataTypeConversion  OutDataTypeStr=single  SaturateOnIntegerOverflow=off  RndMeth=Floor
  Data Type Conversion1 : DataTypeConversion  OutDataTypeStr=single  SaturateOnIntegerOverflow=off  RndMeth=Floor
  Trajectory Time : Constant  Value=0.5  OutDataTypeStr=single
  current Target : Constant  Value=0.3342925916020326
  jointposition : Constant  Value=0  OutDataTypeStr=single
  jointvelocity : Constant  Value=0  OutDataTypeStr=single
  vref : Constant  Value=0  OutDataTypeStr=single
  Targets : Outport
  wires:
  Data Type Conversion1/1 -> Bus Creator/5
  Trajectory Time/1 -> Bus Creator/1
  jointposition/1 -> Bus Creator/2
  current Target/1 -> Data Type Conversion/1
  jointvelocity/1 -> Bus Creator/3
  vref/1 -> Data Type Conversion1/1
  Data Type Conversion/1 -> Bus Creator/4  "motorcurrent"
  Bus Creator/1 -> Targets/1
